simulink model "snap_sys_clk_feng"  (R2019a)
settings: Solver=VariableStepDiscrete  StartTime=0.0  StopTime=10.0  RelTol=1e-3
undefined symbols (not defined in the file): datetime, posixtime
libraries: xbsIndex_r4 x5252, casper_library_misc x69, xps_library x6, casper_library_delays x3
(part 15 of 45)

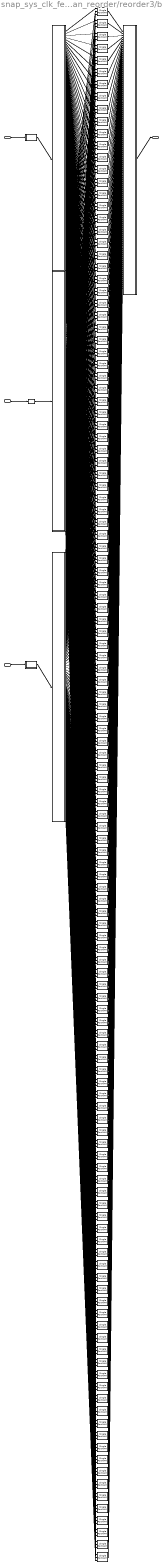
== system snap_sys_clk_feng/chan_reorder/reorder3/buf0 ==
  addr : Inport
  din : Inport  Port=2
  we : Inport  Port=3
  bram{0..127} (128 alike) : xbsIndex_r4/Single Port RAM  depth=16384  initVector=getfield(get_param(gcb, 'UserData'), 'initVector')  distributed_mem=Block RAM  write_mode=Read Before Write  rst=off  init_reg=0  en=off  latency=2  optimize=Speed  dbl_ovrd=off  block_type=spram
  ddin : xbsIndex_r4/Delay  rst=off  infoeditControl=Selection of Reset will increase slice count due to use of real FFs and instead of SRLs  en=off  latency=2  reg_retiming=on  dbl_ovrd=off  block_type=delay
  debus_addr : Subsystem  AncestorBlock=casper_library_flow_control/bus_expand  mask(bus_expand){mode=divisions of equal size, outputNum=128, outputWidth=[14 14 14 14 14 14 14 14 14 14 14 14 14 14 14 14 14 14 14 14 14 14 14 14 14 14 14 14 14 14 14 14 14 14 14 14 14 14 14 14 14 14 14 14 14 14 14 14 14 14 14 14 14 14 14 14 14 14 14 14 14 14 14 14 14 14 14 14 14 14 14 14 14 14 14 14 14 14 14 14 14 14 14 14 14 14 14 14 14 14 14 14 14 14 14 14 14 14 14 14 14 14 14 14 14 14 14 14 14 14 14 14 14 14 14 14 14 14 14 14 14 14 14 14 14 14 14 14], outputBinaryPt=[0 0 0 0 0 0 0 0 0 0 0 0 0 0 0 0 0 0 0 0 0 0 0 0 0 0 0 0 0 0 0 0 0 0 0 0 0 0 0 0 0 0 0 0 0 0 0 0 0 0 0 0 0 0 0 0 0 0 0 0 0 0 0 0 0 0 0 0 0 0 0 0 0 0 0 0 0 0 0 0 0 0 0 0 0 0 0 0 0 0 0 0 0 0 0 0 0 0 0 0 0 0 0 0 0 0 0 0 0 0 0 0 0 0 0 0 0 0 0 0 0 0 0 0 0 0 0 0], outputArithmeticType=[0 0 0 0 0 0 0 0 0 0 0 0 0 0 0 0 0 0 0 0 0 0 0 0 0 0 0 0 0 0 0 0 0 0 0 0 0 0 0 0 0 0 0 0 0 0 0 0 0 0 0 0 0 0 0 0 0 0 0 0 0 0 0 0 0 0 0 0 0 0 0 0 0 0 0 0 0 0 0 0 0 0 0 0 0 0 0 0 0 0 0 0 0 0 0 0 0 0 0 0 0 0 0 0 0 0 0 0 0 0 0 0 0 0 0 0 0 0 0 0 0 0 0 0 0 0 0 0], show_format=on, outputToWorkspace=off, variablePrefix=, outputToModelAsWell=on}
      mask prompts: outputNum "Number of outputs:"; outputWidth "Output width:"; outputBinaryPt "Output binary point position:"; outputArithmeticType "Output arithmetic type (ufix=0, fix=1, bool=2):"; show_format "Print format string?"; outputToWorkspace "Output to workspace?"; variablePrefix "Variable name prefix:"; outputToModelAsWell "Output to model as well?"
      mask help:
      | Expands a 'bus' made using a bus_create or Xilinx
      | concat block.
      | The input will be divided into the specified number
      | of outputs with the specified arithmetic types.
      | Divisions are made from most significant bit.
      mask init: same as snap_sys_clk_feng/corr/bus_expand
      settings: AttributesFormatString=128 outputs: uf14.0,uf14.0,uf14.0,uf14.0,uf14.0,uf14.0,uf14.0,uf14.0,uf14.0,uf14.0,uf14.0,uf14.0,uf14.0,uf14.0,uf14.0,uf14.0,uf14.0,uf14.0,uf14.0,uf14.0,uf14.0,uf14.0,uf14.0,uf14.0,uf14.0,uf14.0,uf14.0,uf14.0,uf14.0,uf14.0,uf14.0,uf14.0,uf14.0,uf14.0,uf14.0,uf14.0,uf14.0,uf14.0,uf14.0,uf14.0,uf14.0,uf14.0,uf14.0,uf14.0,uf14.0,uf14.0,uf14.0,uf14.0,uf14.0,uf14.0,uf14.0,uf14.0,uf14.0,uf14.0,uf14.0,uf14.0,uf14.0,uf14.0,uf14.0,uf14.0,uf14.0,uf14.0,uf14.0,uf14.0,uf14.0,uf14.0,uf14.0,uf14.0,uf14.0,uf14.0,uf14.0,uf14.0,uf14.0,uf14.0,uf14.0,uf14.0,uf14.0,uf14.0,uf14.0,uf14.0,uf14.0,uf14.0,uf14.0,uf14.0,uf14.0,uf14.0,uf14.0,uf14.0,uf14.0,uf14.0,uf14.0,uf14.0,uf14.0,uf14.0,uf14.0,uf14.0,uf14.0,uf14.0,uf14.0,uf14.0,uf14.0,uf14.0,uf14.0,uf14.0,uf14.0,uf14.0,uf14.0,uf14.0,uf14.0,uf14.0,uf14.0,uf14.0,uf14.0,uf14.0,uf14.0,uf14.0,uf14.0,uf14.0,uf14.0,uf14.0,uf14.0,uf14.0,uf14.0,uf14.0,uf14.0,uf14.0,uf14.0,uf14.0,
      mask TypeOptions mode: divisions of equal size | divisions of arbitrary size
      mask Callback mode: bus_expand_callback();
      mask Callback outputWidth: bus_expand_callback();
      mask Callback outputToWorkspace: bus_expand_callback();
  debus_din : Subsystem  AncestorBlock=casper_library_flow_control/bus_expand  mask(bus_expand){mode=divisions of arbitrary size, outputNum=1, outputWidth=[1 1 1 1 1 1 1 1 1 1 1 1 1 1 1 1 1 1 1 1 1 1 1 1 1 1 1 1 1 1 1 1 1 1 1 1 1 1 1 1 1 1 1 1 1 1 1 1 1 1 1 1 1 1 1 1 1 1 1 1 1 1 1 1 1 1 1 1 1 1 1 1 1 1 1 1 1 1 1 1 1 1 1 1 1 1 1 1 1 1 1 1 1 1 1 1 1 1 1 1 1 1 1 1 1 1 1 1 1 1 1 1 1 1 1 1 1 1 1 1 1 1 1 1 1 1 1 1], outputBinaryPt=[0 0 0 0 0 0 0 0 0 0 0 0 0 0 0 0 0 0 0 0 0 0 0 0 0 0 0 0 0 0 0 0 0 0 0 0 0 0 0 0 0 0 0 0 0 0 0 0 0 0 0 0 0 0 0 0 0 0 0 0 0 0 0 0 0 0 0 0 0 0 0 0 0 0 0 0 0 0 0 0 0 0 0 0 0 0 0 0 0 0 0 0 0 0 0 0 0 0 0 0 0 0 0 0 0 0 0 0 0 0 0 0 0 0 0 0 0 0 0 0 0 0 0 0 0 0 0 0], outputArithmeticType=[0 0 0 0 0 0 0 0 0 0 0 0 0 0 0 0 0 0 0 0 0 0 0 0 0 0 0 0 0 0 0 0 0 0 0 0 0 0 0 0 0 0 0 0 0 0 0 0 0 0 0 0 0 0 0 0 0 0 0 0 0 0 0 0 0 0 0 0 0 0 0 0 0 0 0 0 0 0 0 0 0 0 0 0 0 0 0 0 0 0 0 0 0 0 0 0 0 0 0 0 0 0 0 0 0 0 0 0 0 0 0 0 0 0 0 0 0 0 0 0 0 0 0 0 0 0 0 0], show_format=on, outputToWorkspace=off, variablePrefix=, outputToModelAsWell=on}
      mask prompts: outputNum "Number of outputs:"; outputWidth "Output width [msb ... lsb]:"; outputBinaryPt "Output binary point position [msb ... lsb]:"; outputArithmeticType "Output arithmetic type (ufix=0, fix=1, bool=2) [msb ... lsb]:"; show_format "Print format string?"; outputToWorkspace "Output to workspace?"; variablePrefix "Variable name prefix:"; outputToModelAsWell "Output to model as well?"
      mask help:
      | Expands a 'bus' made using a bus_create or Xilinx
      | concat block.
      | The input will be divided into the specified number
      | of outputs with the specified arithmetic types.
      | Divisions are made from most significant bit.
      mask init: same as snap_sys_clk_feng/corr/bus_expand
      settings: AttributesFormatString=128 outputs: uf1.0,uf1.0,uf1.0,uf1.0,uf1.0,uf1.0,uf1.0,uf1.0,uf1.0,uf1.0,uf1.0,uf1.0,uf1.0,uf1.0,uf1.0,uf1.0,uf1.0,uf1.0,uf1.0,uf1.0,uf1.0,uf1.0,uf1.0,uf1.0,uf1.0,uf1.0,uf1.0,uf1.0,uf1.0,uf1.0,uf1.0,uf1.0,uf1.0,uf1.0,uf1.0,uf1.0,uf1.0,uf1.0,uf1.0,uf1.0,uf1.0,uf1.0,uf1.0,uf1.0,uf1.0,uf1.0,uf1.0,uf1.0,uf1.0,uf1.0,uf1.0,uf1.0,uf1.0,uf1.0,uf1.0,uf1.0,uf1.0,uf1.0,uf1.0,uf1.0,uf1.0,uf1.0,uf1.0,uf1.0,uf1.0,uf1.0,uf1.0,uf1.0,uf1.0,uf1.0,uf1.0,uf1.0,uf1.0,uf1.0,uf1.0,uf1.0,uf1.0,uf1.0,uf1.0,uf1.0,uf1.0,uf1.0,uf1.0,uf1.0,uf1.0,uf1.0,uf1.0,uf1.0,uf1.0,uf1.0,uf1.0,uf1.0,uf1.0,uf1.0,uf1.0,uf1.0,uf1.0,uf1.0,uf1.0,uf1.0,uf1.0,uf1.0,uf1.0,uf1.0,uf1.0,uf1.0,uf1.0,uf1.0,uf1.0,uf1.0,uf1.0,uf1.0,uf1.0,uf1.0,uf1.0,uf1.0,uf1.0,uf1.0,uf1.0,uf1.0,uf1.0,uf1.0,uf1.0,uf1.0,uf1.0,uf1.0,uf1.0,uf1.0,
      mask TypeOptions mode: divisions of equal size | divisions of arbitrary size
      mask Callback mode: bus_expand_callback();
      mask Callback outputWidth: bus_expand_callback();
      mask Callback outputToWorkspace: bus_expand_callback();
  debus_we : Subsystem  AncestorBlock=casper_library_flow_control/bus_expand  mask(bus_expand){mode=divisions of equal size, outputNum=128, outputWidth=[1 1 1 1 1 1 1 1 1 1 1 1 1 1 1 1 1 1 1 1 1 1 1 1 1 1 1 1 1 1 1 1 1 1 1 1 1 1 1 1 1 1 1 1 1 1 1 1 1 1 1 1 1 1 1 1 1 1 1 1 1 1 1 1 1 1 1 1 1 1 1 1 1 1 1 1 1 1 1 1 1 1 1 1 1 1 1 1 1 1 1 1 1 1 1 1 1 1 1 1 1 1 1 1 1 1 1 1 1 1 1 1 1 1 1 1 1 1 1 1 1 1 1 1 1 1 1 1], outputBinaryPt=[0 0 0 0 0 0 0 0 0 0 0 0 0 0 0 0 0 0 0 0 0 0 0 0 0 0 0 0 0 0 0 0 0 0 0 0 0 0 0 0 0 0 0 0 0 0 0 0 0 0 0 0 0 0 0 0 0 0 0 0 0 0 0 0 0 0 0 0 0 0 0 0 0 0 0 0 0 0 0 0 0 0 0 0 0 0 0 0 0 0 0 0 0 0 0 0 0 0 0 0 0 0 0 0 0 0 0 0 0 0 0 0 0 0 0 0 0 0 0 0 0 0 0 0 0 0 0 0], outputArithmeticType=[2 2 2 2 2 2 2 2 2 2 2 2 2 2 2 2 2 2 2 2 2 2 2 2 2 2 2 2 2 2 2 2 2 2 2 2 2 2 2 2 2 2 2 2 2 2 2 2 2 2 2 2 2 2 2 2 2 2 2 2 2 2 2 2 2 2 2 2 2 2 2 2 2 2 2 2 2 2 2 2 2 2 2 2 2 2 2 2 2 2 2 2 2 2 2 2 2 2 2 2 2 2 2 2 2 2 2 2 2 2 2 2 2 2 2 2 2 2 2 2 2 2 2 2 2 2 2 2], show_format=on, outputToWorkspace=off, variablePrefix=, outputToModelAsWell=on}
      mask prompts: outputNum "Number of outputs:"; outputWidth "Output width:"; outputBinaryPt "Output binary point position:"; outputArithmeticType "Output arithmetic type (ufix=0, fix=1, bool=2):"; show_format "Print format string?"; outputToWorkspace "Output to workspace?"; variablePrefix "Variable name prefix:"; outputToModelAsWell "Output to model as well?"
      mask help:
      | Expands a 'bus' made using a bus_create or Xilinx
      | concat block.
      | The input will be divided into the specified number
      | of outputs with the specified arithmetic types.
      | Divisions are made from most significant bit.
      mask init: same as snap_sys_clk_feng/corr/bus_expand
      settings: AttributesFormatString=128 outputs: b,b,b,b,b,b,b,b,b,b,b,b,b,b,b,b,b,b,b,b,b,b,b,b,b,b,b,b,b,b,b,b,b,b,b,b,b,b,b,b,b,b,b,b,b,b,b,b,b,b,b,b,b,b,b,b,b,b,b,b,b,b,b,b,b,b,b,b,b,b,b,b,b,b,b,b,b,b,b,b,b,b,b,b,b,b,b,b,b,b,b,b,b,b,b,b,b,b,b,b,b,b,b,b,b,b,b,b,b,b,b,b,b,b,b,b,b,b,b,b,b,b,b,b,b,b,b,b,
      mask TypeOptions mode: divisions of equal size | divisions of arbitrary size
      mask Callback mode: bus_expand_callback();
      mask Callback outputWidth: bus_expand_callback();
      mask Callback outputToWorkspace: bus_expand_callback();
  din_bussify : Subsystem  AncestorBlock=casper_library_flow_control/bus_create  mask(bus_create){inputNum=128}
      mask prompts: inputNum "Number of inputs:"
      mask init:
      | bus_create_init(gcb,...
      |     'inputNum', inputNum);
  rep_addr : Subsystem  AncestorBlock=casper_library_bus/bus_replicate  mask(bus_replicate){replication=128, csp_latency=2, misc=off, implementation=core}
      mask prompts: replication "replication factor"; csp_latency "latency"; misc "misc support"; implementation "delay implementation"
      mask help: Output bus formed by replicating input bus a number of times
      mask init:
      | bus_replicate_init(gcb, ...
      |     'replication', replication, ...
      |     'csp_latency', csp_latency, ...
      |     'implementation', implementation, ...
      |     'misc', misc);
      mask TypeOptions implementation: core | behavioral
  rep_we : Subsystem  AncestorBlock=casper_library_bus/bus_replicate  mask(bus_replicate){replication=128, csp_latency=2, misc=off, implementation=core}
      mask prompts: replication "replication factor"; csp_latency "latency"; misc "misc support"; implementation "delay implementation"
      mask help: Output bus formed by replicating input bus a number of times
      mask init:
      | bus_replicate_init(gcb, ...
      |     'replication', replication, ...
      |     'csp_latency', csp_latency, ...
      |     'implementation', implementation, ...
      |     'misc', misc);
      mask TypeOptions implementation: core | behavioral
  dout : Outport
  wires:
  addr/1 -> rep_addr/1(in)
  din/1 -> ddin/1
  we/1 -> rep_we/1(in)
  rep_addr/1(out) -> debus_addr/1(bus_in)
  ddin/1 -> debus_din/1(bus_in)
  rep_we/1(out) -> debus_we/1(bus_in)
  debus_addr/1(msb_out128) -> bram0/1
  debus_din/1(msb_out128) -> bram0/2
  debus_we/1(msb_out128) -> bram0/3
  debus_addr/2(out127) -> bram1/1
  debus_din/2(out127) -> bram1/2
  debus_we/2(out127) -> bram1/3
  debus_addr/3(out126) -> bram2/1
  debus_din/3(out126) -> bram2/2
  debus_we/3(out126) -> bram2/3
  debus_addr/4(out125) -> bram3/1
  debus_din/4(out125) -> bram3/2
  debus_we/4(out125) -> bram3/3
  debus_addr/5(out124) -> bram4/1
  debus_din/5(out124) -> bram4/2
  debus_we/5(out124) -> bram4/3
  debus_addr/6(out123) -> bram5/1
  debus_din/6(out123) -> bram5/2
  debus_we/6(out123) -> bram5/3
  debus_addr/7(out122) -> bram6/1
  debus_din/7(out122) -> bram6/2
  debus_we/7(out122) -> bram6/3
  debus_addr/8(out121) -> bram7/1
  debus_din/8(out121) -> bram7/2
  debus_we/8(out121) -> bram7/3
  debus_addr/9(out120) -> bram8/1
  debus_din/9(out120) -> bram8/2
  debus_we/9(out120) -> bram8/3
  debus_addr/10(out119) -> bram9/1
  debus_din/10(out119) -> bram9/2
  debus_we/10(out119) -> bram9/3
  debus_addr/11(out118) -> bram10/1
  debus_din/11(out118) -> bram10/2
  debus_we/11(out118) -> bram10/3
  debus_addr/12(out117) -> bram11/1
  debus_din/12(out117) -> bram11/2
  debus_we/12(out117) -> bram11/3
  debus_addr/13(out116) -> bram12/1
  debus_din/13(out116) -> bram12/2
  debus_we/13(out116) -> bram12/3
  debus_addr/14(out115) -> bram13/1
  debus_din/14(out115) -> bram13/2
  debus_we/14(out115) -> bram13/3
  debus_addr/15(out114) -> bram14/1
  debus_din/15(out114) -> bram14/2
  debus_we/15(out114) -> bram14/3
  debus_addr/16(out113) -> bram15/1
  debus_din/16(out113) -> bram15/2
  debus_we/16(out113) -> bram15/3
  debus_addr/17(out112) -> bram16/1
  debus_din/17(out112) -> bram16/2
  debus_we/17(out112) -> bram16/3
  debus_addr/18(out111) -> bram17/1
  debus_din/18(out111) -> bram17/2
  debus_we/18(out111) -> bram17/3
  debus_addr/19(out110) -> bram18/1
  debus_din/19(out110) -> bram18/2
  debus_we/19(out110) -> bram18/3
  debus_addr/20(out109) -> bram19/1
  debus_din/20(out109) -> bram19/2
  debus_we/20(out109) -> bram19/3
  debus_addr/21(out108) -> bram20/1
  debus_din/21(out108) -> bram20/2
  debus_we/21(out108) -> bram20/3
  debus_addr/22(out107) -> bram21/1
  debus_din/22(out107) -> bram21/2
  debus_we/22(out107) -> bram21/3
  debus_addr/23(out106) -> bram22/1
  debus_din/23(out106) -> bram22/2
  debus_we/23(out106) -> bram22/3
  debus_addr/24(out105) -> bram23/1
  debus_din/24(out105) -> bram23/2
  debus_we/24(out105) -> bram23/3
  debus_addr/25(out104) -> bram24/1
  debus_din/25(out104) -> bram24/2
  debus_we/25(out104) -> bram24/3
  debus_addr/26(out103) -> bram25/1
  debus_din/26(out103) -> bram25/2
  debus_we/26(out103) -> bram25/3
  debus_addr/27(out102) -> bram26/1
  debus_din/27(out102) -> bram26/2
  debus_we/27(out102) -> bram26/3
  debus_addr/28(out101) -> bram27/1
  debus_din/28(out101) -> bram27/2
  debus_we/28(out101) -> bram27/3
  debus_addr/29(out100) -> bram28/1
  debus_din/29(out100) -> bram28/2
  debus_we/29(out100) -> bram28/3
  debus_addr/30(out99) -> bram29/1
  debus_din/30(out99) -> bram29/2
  debus_we/30(out99) -> bram29/3
  debus_addr/31(out98) -> bram30/1
  debus_din/31(out98) -> bram30/2
  debus_we/31(out98) -> bram30/3
  debus_addr/32(out97) -> bram31/1
  debus_din/32(out97) -> bram31/2
  debus_we/32(out97) -> bram31/3
  debus_addr/33(out96) -> bram32/1
  debus_din/33(out96) -> bram32/2
  debus_we/33(out96) -> bram32/3
  debus_addr/34(out95) -> bram33/1
  debus_din/34(out95) -> bram33/2
  debus_we/34(out95) -> bram33/3
  debus_addr/35(out94) -> bram34/1
  debus_din/35(out94) -> bram34/2
  debus_we/35(out94) -> bram34/3
  debus_addr/36(out93) -> bram35/1
  debus_din/36(out93) -> bram35/2
  debus_we/36(out93) -> bram35/3
  debus_addr/37(out92) -> bram36/1
  debus_din/37(out92) -> bram36/2
  debus_we/37(out92) -> bram36/3
  debus_addr/38(out91) -> bram37/1
  debus_din/38(out91) -> bram37/2
  debus_we/38(out91) -> bram37/3
  debus_addr/39(out90) -> bram38/1
  debus_din/39(out90) -> bram38/2
  debus_we/39(out90) -> bram38/3
  debus_addr/40(out89) -> bram39/1
  debus_din/40(out89) -> bram39/2
  debus_we/40(out89) -> bram39/3
  debus_addr/41(out88) -> bram40/1
  debus_din/41(out88) -> bram40/2
  debus_we/41(out88) -> bram40/3
  debus_addr/42(out87) -> bram41/1
  debus_din/42(out87) -> bram41/2
  debus_we/42(out87) -> bram41/3
  debus_addr/43(out86) -> bram42/1
  debus_din/43(out86) -> bram42/2
  debus_we/43(out86) -> bram42/3
  debus_addr/44(out85) -> bram43/1
  debus_din/44(out85) -> bram43/2
  debus_we/44(out85) -> bram43/3
  debus_addr/45(out84) -> bram44/1
  debus_din/45(out84) -> bram44/2
  debus_we/45(out84) -> bram44/3
  debus_addr/46(out83) -> bram45/1
  debus_din/46(out83) -> bram45/2
  debus_we/46(out83) -> bram45/3
  debus_addr/47(out82) -> bram46/1
  debus_din/47(out82) -> bram46/2
  debus_we/47(out82) -> bram46/3
  debus_addr/48(out81) -> bram47/1
  debus_din/48(out81) -> bram47/2
  debus_we/48(out81) -> bram47/3
  debus_addr/49(out80) -> bram48/1
  debus_din/49(out80) -> bram48/2
  debus_we/49(out80) -> bram48/3
  debus_addr/50(out79) -> bram49/1
  debus_din/50(out79) -> bram49/2
  debus_we/50(out79) -> bram49/3
  debus_addr/51(out78) -> bram50/1
  debus_din/51(out78) -> bram50/2
  debus_we/51(out78) -> bram50/3
  debus_addr/52(out77) -> bram51/1
  debus_din/52(out77) -> bram51/2
  debus_we/52(out77) -> bram51/3
  debus_addr/53(out76) -> bram52/1
  debus_din/53(out76) -> bram52/2
  debus_we/53(out76) -> bram52/3
  debus_addr/54(out75) -> bram53/1
  debus_din/54(out75) -> bram53/2
  debus_we/54(out75) -> bram53/3
  debus_addr/55(out74) -> bram54/1
  debus_din/55(out74) -> bram54/2
  debus_we/55(out74) -> bram54/3
  debus_addr/56(out73) -> bram55/1
  debus_din/56(out73) -> bram55/2
  debus_we/56(out73) -> bram55/3
  debus_addr/57(out72) -> bram56/1
  debus_din/57(out72) -> bram56/2
  debus_we/57(out72) -> bram56/3
  debus_addr/58(out71) -> bram57/1
  debus_din/58(out71) -> bram57/2
  debus_we/58(out71) -> bram57/3
  debus_addr/59(out70) -> bram58/1
  debus_din/59(out70) -> bram58/2
  debus_we/59(out70) -> bram58/3
  debus_addr/60(out69) -> bram59/1
  debus_din/60(out69) -> bram59/2
  debus_we/60(out69) -> bram59/3
  debus_addr/61(out68) -> bram60/1
  debus_din/61(out68) -> bram60/2
  debus_we/61(out68) -> bram60/3
  debus_addr/62(out67) -> bram61/1
  debus_din/62(out67) -> bram61/2
  debus_we/62(out67) -> bram61/3
  debus_addr/63(out66) -> bram62/1
  debus_din/63(out66) -> bram62/2
  debus_we/63(out66) -> bram62/3
  debus_addr/64(out65) -> bram63/1
  debus_din/64(out65) -> bram63/2
  debus_we/64(out65) -> bram63/3
  debus_addr/65(out64) -> bram64/1
  debus_din/65(out64) -> bram64/2
  debus_we/65(out64) -> bram64/3
  debus_addr/66(out63) -> bram65/1
  debus_din/66(out63) -> bram65/2
  debus_we/66(out63) -> bram65/3
  debus_addr/67(out62) -> bram66/1
  debus_din/67(out62) -> bram66/2
  debus_we/67(out62) -> bram66/3
  debus_addr/68(out61) -> bram67/1
  debus_din/68(out61) -> bram67/2
  debus_we/68(out61) -> bram67/3
  debus_addr/69(out60) -> bram68/1
  debus_din/69(out60) -> bram68/2
  debus_we/69(out60) -> bram68/3
  debus_addr/70(out59) -> bram69/1
  debus_din/70(out59) -> bram69/2
  debus_we/70(out59) -> bram69/3
  debus_addr/71(out58) -> bram70/1
  debus_din/71(out58) -> bram70/2
  debus_we/71(out58) -> bram70/3
  debus_addr/72(out57) -> bram71/1
  debus_din/72(out57) -> bram71/2
  debus_we/72(out57) -> bram71/3
  debus_addr/73(out56) -> bram72/1
  debus_din/73(out56) -> bram72/2
  debus_we/73(out56) -> bram72/3
  debus_addr/74(out55) -> bram73/1
  debus_din/74(out55) -> bram73/2
  debus_we/74(out55) -> bram73/3
  debus_addr/75(out54) -> bram74/1
  debus_din/75(out54) -> bram74/2
  debus_we/75(out54) -> bram74/3
  debus_addr/76(out53) -> bram75/1
  debus_din/76(out53) -> bram75/2
  debus_we/76(out53) -> bram75/3
  debus_addr/77(out52) -> bram76/1
  debus_din/77(out52) -> bram76/2
  debus_we/77(out52) -> bram76/3
  debus_addr/78(out51) -> bram77/1
  debus_din/78(out51) -> bram77/2
  debus_we/78(out51) -> bram77/3
  debus_addr/79(out50) -> bram78/1
  debus_din/79(out50) -> bram78/2
  debus_we/79(out50) -> bram78/3
  debus_addr/80(out49) -> bram79/1
  debus_din/80(out49) -> bram79/2
  debus_we/80(out49) -> bram79/3
  debus_addr/81(out48) -> bram80/1
  debus_din/81(out48) -> bram80/2
  debus_we/81(out48) -> bram80/3
  debus_addr/82(out47) -> bram81/1
  debus_din/82(out47) -> bram81/2
  debus_we/82(out47) -> bram81/3
  debus_addr/83(out46) -> bram82/1
  debus_din/83(out46) -> bram82/2
  debus_we/83(out46) -> bram82/3
  debus_addr/84(out45) -> bram83/1
  debus_din/84(out45) -> bram83/2
  debus_we/84(out45) -> bram83/3
  debus_addr/85(out44) -> bram84/1
  debus_din/85(out44) -> bram84/2
  debus_we/85(out44) -> bram84/3
  debus_addr/86(out43) -> bram85/1
  debus_din/86(out43) -> bram85/2
  debus_we/86(out43) -> bram85/3
  debus_addr/87(out42) -> bram86/1
  debus_din/87(out42) -> bram86/2
  debus_we/87(out42) -> bram86/3
  debus_addr/88(out41) -> bram87/1
  debus_din/88(out41) -> bram87/2
  debus_we/88(out41) -> bram87/3
  debus_addr/89(out40) -> bram88/1
  debus_din/89(out40) -> bram88/2
  debus_we/89(out40) -> bram88/3
  debus_addr/90(out39) -> bram89/1
  debus_din/90(out39) -> bram89/2
  debus_we/90(out39) -> bram89/3
  debus_addr/91(out38) -> bram90/1
  debus_din/91(out38) -> bram90/2
  debus_we/91(out38) -> bram90/3
  debus_addr/92(out37) -> bram91/1
  debus_din/92(out37) -> bram91/2
  debus_we/92(out37) -> bram91/3
  debus_addr/93(out36) -> bram92/1
  debus_din/93(out36) -> bram92/2
  debus_we/93(out36) -> bram92/3
  debus_addr/94(out35) -> bram93/1
  debus_din/94(out35) -> bram93/2
  debus_we/94(out35) -> bram93/3
  debus_addr/95(out34) -> bram94/1
  debus_din/95(out34) -> bram94/2
  debus_we/95(out34) -> bram94/3
  debus_addr/96(out33) -> bram95/1
  debus_din/96(out33) -> bram95/2
  debus_we/96(out33) -> bram95/3
  debus_addr/97(out32) -> bram96/1
  debus_din/97(out32) -> bram96/2
  debus_we/97(out32) -> bram96/3
  debus_addr/98(out31) -> bram97/1
  debus_din/98(out31) -> bram97/2
  debus_we/98(out31) -> bram97/3
  debus_addr/99(out30) -> bram98/1
  debus_din/99(out30) -> bram98/2
  debus_we/99(out30) -> bram98/3
  debus_addr/100(out29) -> bram99/1
  debus_din/100(out29) -> bram99/2
  debus_we/100(out29) -> bram99/3
  debus_addr/101(out28) -> bram100/1
  debus_din/101(out28) -> bram100/2
  debus_we/101(out28) -> bram100/3
  debus_addr/102(out27) -> bram101/1
  debus_din/102(out27) -> bram101/2
  debus_we/102(out27) -> bram101/3
  debus_addr/103(out26) -> bram102/1
  debus_din/103(out26) -> bram102/2
  debus_we/103(out26) -> bram102/3
  debus_addr/104(out25) -> bram103/1
  debus_din/104(out25) -> bram103/2
  debus_we/104(out25) -> bram103/3
  debus_addr/105(out24) -> bram104/1
  debus_din/105(out24) -> bram104/2
  debus_we/105(out24) -> bram104/3
  debus_addr/106(out23) -> bram105/1
  debus_din/106(out23) -> bram105/2
  debus_we/106(out23) -> bram105/3
  debus_addr/107(out22) -> bram106/1
  debus_din/107(out22) -> bram106/2
  debus_we/107(out22) -> bram106/3
  debus_addr/108(out21) -> bram107/1
  debus_din/108(out21) -> bram107/2
  debus_we/108(out21) -> bram107/3
  debus_addr/109(out20) -> bram108/1
  debus_din/109(out20) -> bram108/2
  debus_we/109(out20) -> bram108/3
  debus_addr/110(out19) -> bram109/1
  debus_din/110(out19) -> bram109/2
  debus_we/110(out19) -> bram109/3
  debus_addr/111(out18) -> bram110/1
  debus_din/111(out18) -> bram110/2
  debus_we/111(out18) -> bram110/3
  debus_addr/112(out17) -> bram111/1
  debus_din/112(out17) -> bram111/2
  debus_we/112(out17) -> bram111/3
  debus_addr/113(out16) -> bram112/1
  debus_din/113(out16) -> bram112/2
  debus_we/113(out16) -> bram112/3
  debus_addr/114(out15) -> bram113/1
  debus_din/114(out15) -> bram113/2
  debus_we/114(out15) -> bram113/3
  debus_addr/115(out14) -> bram114/1
  debus_din/115(out14) -> bram114/2
  debus_we/115(out14) -> bram114/3
  debus_addr/116(out13) -> bram115/1
  debus_din/116(out13) -> bram115/2
  debus_we/116(out13) -> bram115/3
  debus_addr/117(out12) -> bram116/1
  debus_din/117(out12) -> bram116/2
  debus_we/117(out12) -> bram116/3
  debus_addr/118(out11) -> bram117/1
  debus_din/118(out11) -> bram117/2
  debus_we/118(out11) -> bram117/3
  debus_addr/119(out10) -> bram118/1
  debus_din/119(out10) -> bram118/2
  debus_we/119(out10) -> bram118/3
  debus_addr/120(out9) -> bram119/1
  debus_din/120(out9) -> bram119/2
  debus_we/120(out9) -> bram119/3
  debus_addr/121(out8) -> bram120/1
  debus_din/121(out8) -> bram120/2
  debus_we/121(out8) -> bram120/3
  debus_addr/122(out7) -> bram121/1
  debus_din/122(out7) -> bram121/2
  debus_we/122(out7) -> bram121/3
  debus_addr/123(out6) -> bram122/1
  debus_din/123(out6) -> bram122/2
  debus_we/123(out6) -> bram122/3
  debus_addr/124(out5) -> bram123/1
  debus_din/124(out5) -> bram123/2
  debus_we/124(out5) -> bram123/3
  debus_addr/125(out4) -> bram124/1
  debus_din/125(out4) -> bram124/2
  debus_we/125(out4) -> bram124/3
  debus_addr/126(out3) -> bram125/1
  debus_din/126(out3) -> bram125/2
  debus_we/126(out3) -> bram125/3
  debus_addr/127(out2) -> bram126/1
  debus_din/127(out2) -> bram126/2
  debus_we/127(out2) -> bram126/3
  debus_addr/128(lsb_out1) -> bram127/1
  debus_din/128(lsb_out1) -> bram127/2
  debus_we/128(lsb_out1) -> bram127/3
  bram0/1 -> din_bussify/1(in1)
  bram1/1 -> din_bussify/2(in2)
  bram2/1 -> din_bussify/3(in3)
  bram3/1 -> din_bussify/4(in4)
  bram4/1 -> din_bussify/5(in5)
  bram5/1 -> din_bussify/6(in6)
  bram6/1 -> din_bussify/7(in7)
  bram7/1 -> din_bussify/8(in8)
  bram8/1 -> din_bussify/9(in9)
  bram9/1 -> din_bussify/10(in10)
  bram10/1 -> din_bussify/11(in11)
  bram11/1 -> din_bussify/12(in12)
  bram12/1 -> din_bussify/13(in13)
  bram13/1 -> din_bussify/14(in14)
  bram14/1 -> din_bussify/15(in15)
  bram15/1 -> din_bussify/16(in16)
  bram16/1 -> din_bussify/17(in17)
  bram17/1 -> din_bussify/18(in18)
  bram18/1 -> din_bussify/19(in19)
  bram19/1 -> din_bussify/20(in20)
  bram20/1 -> din_bussify/21(in21)
  bram21/1 -> din_bussify/22(in22)
  bram22/1 -> din_bussify/23(in23)
  bram23/1 -> din_bussify/24(in24)
  bram24/1 -> din_bussify/25(in25)
  bram25/1 -> din_bussify/26(in26)
  bram26/1 -> din_bussify/27(in27)
  bram27/1 -> din_bussify/28(in28)
  bram28/1 -> din_bussify/29(in29)
  bram29/1 -> din_bussify/30(in30)
  bram30/1 -> din_bussify/31(in31)
  bram31/1 -> din_bussify/32(in32)
  bram32/1 -> din_bussify/33(in33)
  bram33/1 -> din_bussify/34(in34)
  bram34/1 -> din_bussify/35(in35)
  bram35/1 -> din_bussify/36(in36)
  bram36/1 -> din_bussify/37(in37)
  bram37/1 -> din_bussify/38(in38)
  bram38/1 -> din_bussify/39(in39)
  bram39/1 -> din_bussify/40(in40)
  bram40/1 -> din_bussify/41(in41)
  bram41/1 -> din_bussify/42(in42)
  bram42/1 -> din_bussify/43(in43)
  bram43/1 -> din_bussify/44(in44)
  bram44/1 -> din_bussify/45(in45)
  bram45/1 -> din_bussify/46(in46)
  bram46/1 -> din_bussify/47(in47)
  bram47/1 -> din_bussify/48(in48)
  bram48/1 -> din_bussify/49(in49)
  bram49/1 -> din_bussify/50(in50)
  bram50/1 -> din_bussify/51(in51)
  bram51/1 -> din_bussify/52(in52)
  bram52/1 -> din_bussify/53(in53)
  bram53/1 -> din_bussify/54(in54)
  bram54/1 -> din_bussify/55(in55)
  bram55/1 -> din_bussify/56(in56)
  bram56/1 -> din_bussify/57(in57)
  bram57/1 -> din_bussify/58(in58)
  bram58/1 -> din_bussify/59(in59)
  bram59/1 -> din_bussify/60(in60)
  bram60/1 -> din_bussify/61(in61)
  bram61/1 -> din_bussify/62(in62)
  bram62/1 -> din_bussify/63(in63)
  bram63/1 -> din_bussify/64(in64)
  bram64/1 -> din_bussify/65(in65)
  bram65/1 -> din_bussify/66(in66)
  bram66/1 -> din_bussify/67(in67)
  bram67/1 -> din_bussify/68(in68)
  bram68/1 -> din_bussify/69(in69)
  bram69/1 -> din_bussify/70(in70)
  bram70/1 -> din_bussify/71(in71)
  bram71/1 -> din_bussify/72(in72)
  bram72/1 -> din_bussify/73(in73)
  bram73/1 -> din_bussify/74(in74)
  bram74/1 -> din_bussify/75(in75)
  bram75/1 -> din_bussify/76(in76)
  bram76/1 -> din_bussify/77(in77)
  bram77/1 -> din_bussify/78(in78)
  bram78/1 -> din_bussify/79(in79)
  bram79/1 -> din_bussify/80(in80)
  bram80/1 -> din_bussify/81(in81)
  bram81/1 -> din_bussify/82(in82)
  bram82/1 -> din_bussify/83(in83)
  bram83/1 -> din_bussify/84(in84)
  bram84/1 -> din_bussify/85(in85)
  bram85/1 -> din_bussify/86(in86)
  bram86/1 -> din_bussify/87(in87)
  bram87/1 -> din_bussify/88(in88)
  bram88/1 -> din_bussify/89(in89)
  bram89/1 -> din_bussify/90(in90)
  bram90/1 -> din_bussify/91(in91)
  bram91/1 -> din_bussify/92(in92)
  bram92/1 -> din_bussify/93(in93)
  bram93/1 -> din_bussify/94(in94)
  bram94/1 -> din_bussify/95(in95)
  bram95/1 -> din_bussify/96(in96)
  bram96/1 -> din_bussify/97(in97)
  bram97/1 -> din_bussify/98(in98)
  bram98/1 -> din_bussify/99(in99)
  bram99/1 -> din_bussify/100(in100)
  bram100/1 -> din_bussify/101(in101)
  bram101/1 -> din_bussify/102(in102)
  bram102/1 -> din_bussify/103(in103)
  bram103/1 -> din_bussify/104(in104)
  bram104/1 -> din_bussify/105(in105)
  bram105/1 -> din_bussify/106(in106)
  bram106/1 -> din_bussify/107(in107)
  bram107/1 -> din_bussify/108(in108)
  bram108/1 -> din_bussify/109(in109)
  bram109/1 -> din_bussify/110(in110)
  bram110/1 -> din_bussify/111(in111)
  bram111/1 -> din_bussify/112(in112)
  bram112/1 -> din_bussify/113(in113)
  bram113/1 -> din_bussify/114(in114)
  bram114/1 -> din_bussify/115(in115)
  bram115/1 -> din_bussify/116(in116)
  bram116/1 -> din_bussify/117(in117)
  bram117/1 -> din_bussify/118(in118)
  bram118/1 -> din_bussify/119(in119)
  bram119/1 -> din_bussify/120(in120)
  bram120/1 -> din_bussify/121(in121)
  bram121/1 -> din_bussify/122(in122)
  bram122/1 -> din_bussify/123(in123)
  bram123/1 -> din_bussify/124(in124)
  bram124/1 -> din_bussify/125(in125)
  bram125/1 -> din_bussify/126(in126)
  bram126/1 -> din_bussify/127(in127)
  bram127/1 -> din_bussify/128(in128)
  din_bussify/1(bus_out) -> dout/1

== system snap_sys_clk_feng/chan_reorder/reorder3/current_map ==
  addra : Inport
  dina : Inport  Port=2
  wea : Inport  Port=3
  addrb : Inport  Port=4
  dinb : Inport  Port=5
  web : Inport  Port=6
  A_bussify0 : Subsystem  AncestorBlock=casper_library_flow_control/bus_create  mask(bus_create){inputNum=7}
      mask prompts: inputNum "Number of inputs:"
      mask init:
      | bus_create_init(gcb,...
      |     'inputNum', inputNum);
  B_bussify0 : Subsystem  AncestorBlock=casper_library_flow_control/bus_create  mask(bus_create){inputNum=7}
      mask prompts: inputNum "Number of inputs:"
      mask init:
      | bus_create_init(gcb,...
      |     'inputNum', inputNum);
  alsbs_slice : xbsIndex_r4/Slice  nbits=14  boolean_output=off  mode=Lower Bit Location + Width  bit1=0  base1=LSB of Input  bit0=0  base0=LSB of Input  dbl_ovrd=off  block_type=slice
  blsbs_slice : xbsIndex_r4/Slice  nbits=14  boolean_output=off  mode=Lower Bit Location + Width  bit1=0  base1=LSB of Input  bit0=0  base0=LSB of Input  dbl_ovrd=off  block_type=slice
  bram0_{0..6} (7 alike) : xbsIndex_r4/Dual Port RAM  depth=16384  initVector=getfield(get_param(gcb, 'UserData'), 'initVector')  distributed_mem=Block RAM  init_a=0  init_b=0  rst_a=off  rst_b=off  en_a=off  en_b=off  latency=2  write_mode_A=Read Before Write  write_mode_B=Read Before Write  optimize=Speed  dbl_ovrd=off  block_type=dpram
  ddina0 : xbsIndex_r4/Delay  rst=off  infoeditControl=Selection of Reset will increase slice count due to use of real FFs and instead of SRLs  en=off  latency=0  reg_retiming=on  dbl_ovrd=off  block_type=delay
  ddinb0 : xbsIndex_r4/Delay  rst=off  infoeditControl=Selection of Reset will increase slice count due to use of real FFs and instead of SRLs  en=off  latency=0  reg_retiming=on  dbl_ovrd=off  block_type=delay
  debus_addra0 : Subsystem  AncestorBlock=casper_library_flow_control/bus_expand  mask(bus_expand){mode=divisions of equal size, outputNum=7, outputWidth=[14 14 14 14 14 14 14], outputBinaryPt=[0 0 0 0 0 0 0], outputArithmeticType=[0 0 0 0 0 0 0], show_format=on, outputToWorkspace=off, variablePrefix=, outputToModelAsWell=on}
      mask prompts: outputNum "Number of outputs:"; outputWidth "Output width:"; outputBinaryPt "Output binary point position:"; outputArithmeticType "Output arithmetic type (ufix=0, fix=1, bool=2):"; show_format "Print format string?"; outputToWorkspace "Output to workspace?"; variablePrefix "Variable name prefix:"; outputToModelAsWell "Output to model as well?"
      mask help:
      | Expands a 'bus' made using a bus_create or Xilinx
      | concat block.
      | The input will be divided into the specified number
      | of outputs with the specified arithmetic types.
      | Divisions are made from most significant bit.
      mask init: same as snap_sys_clk_feng/corr/bus_expand
      settings: AttributesFormatString=7 outputs: uf14.0,uf14.0,uf14.0,uf14.0,uf14.0,uf14.0,uf14.0,
      mask TypeOptions mode: divisions of equal size | divisions of arbitrary size
      mask Callback mode: bus_expand_callback();
      mask Callback outputWidth: bus_expand_callback();
      mask Callback outputToWorkspace: bus_expand_callback();
  debus_addrb0 : Subsystem  AncestorBlock=casper_library_flow_control/bus_expand  mask(bus_expand){mode=divisions of equal size, outputNum=7, outputWidth=[14 14 14 14 14 14 14], outputBinaryPt=[0 0 0 0 0 0 0], outputArithmeticType=[0 0 0 0 0 0 0], show_format=on, outputToWorkspace=off, variablePrefix=, outputToModelAsWell=on}
      mask prompts: outputNum "Number of outputs:"; outputWidth "Output width:"; outputBinaryPt "Output binary point position:"; outputArithmeticType "Output arithmetic type (ufix=0, fix=1, bool=2):"; show_format "Print format string?"; outputToWorkspace "Output to workspace?"; variablePrefix "Variable name prefix:"; outputToModelAsWell "Output to model as well?"
      mask help:
      | Expands a 'bus' made using a bus_create or Xilinx
      | concat block.
      | The input will be divided into the specified number
      | of outputs with the specified arithmetic types.
      | Divisions are made from most significant bit.
      mask init: same as snap_sys_clk_feng/corr/bus_expand
      settings: AttributesFormatString=7 outputs: uf14.0,uf14.0,uf14.0,uf14.0,uf14.0,uf14.0,uf14.0,
      mask TypeOptions mode: divisions of equal size | divisions of arbitrary size
      mask Callback mode: bus_expand_callback();
      mask Callback outputWidth: bus_expand_callback();
      mask Callback outputToWorkspace: bus_expand_callback();
  debus_dina0 : Subsystem  AncestorBlock=casper_library_flow_control/bus_expand  mask(bus_expand){mode=divisions of arbitrary size, outputNum=1, outputWidth=[2 2 2 2 2 2 2], outputBinaryPt=[0 0 0 0 0 0 0], outputArithmeticType=[0 0 0 0 0 0 0], show_format=on, outputToWorkspace=off, variablePrefix=, outputToModelAsWell=on}
      mask prompts: outputNum "Number of outputs:"; outputWidth "Output width [msb ... lsb]:"; outputBinaryPt "Output binary point position [msb ... lsb]:"; outputArithmeticType "Output arithmetic type (ufix=0, fix=1, bool=2) [msb ... lsb]:"; show_format "Print format string?"; outputToWorkspace "Output to workspace?"; variablePrefix "Variable name prefix:"; outputToModelAsWell "Output to model as well?"
      mask help:
      | Expands a 'bus' made using a bus_create or Xilinx
      | concat block.
      | The input will be divided into the specified number
      | of outputs with the specified arithmetic types.
      | Divisions are made from most significant bit.
      mask init: same as snap_sys_clk_feng/corr/bus_expand
      settings: AttributesFormatString=7 outputs: uf2.0,uf2.0,uf2.0,uf2.0,uf2.0,uf2.0,uf2.0,
      mask TypeOptions mode: divisions of equal size | divisions of arbitrary size
      mask Callback mode: bus_expand_callback();
      mask Callback outputWidth: bus_expand_callback();
      mask Callback outputToWorkspace: bus_expand_callback();
  debus_dinb0 : Subsystem  AncestorBlock=casper_library_flow_control/bus_expand  mask(bus_expand){mode=divisions of arbitrary size, outputNum=1, outputWidth=[2 2 2 2 2 2 2], outputBinaryPt=[0 0 0 0 0 0 0], outputArithmeticType=[0 0 0 0 0 0 0], show_format=on, outputToWorkspace=off, variablePrefix=, outputToModelAsWell=on}
      mask prompts: outputNum "Number of outputs:"; outputWidth "Output width [msb ... lsb]:"; outputBinaryPt "Output binary point position [msb ... lsb]:"; outputArithmeticType "Output arithmetic type (ufix=0, fix=1, bool=2) [msb ... lsb]:"; show_format "Print format string?"; outputToWorkspace "Output to workspace?"; variablePrefix "Variable name prefix:"; outputToModelAsWell "Output to model as well?"
      mask help:
      | Expands a 'bus' made using a bus_create or Xilinx
      | concat block.
      | The input will be divided into the specified number
      | of outputs with the specified arithmetic types.
      | Divisions are made from most significant bit.
      mask init: same as snap_sys_clk_feng/corr/bus_expand
      settings: AttributesFormatString=7 outputs: uf2.0,uf2.0,uf2.0,uf2.0,uf2.0,uf2.0,uf2.0,
      mask TypeOptions mode: divisions of equal size | divisions of arbitrary size
      mask Callback mode: bus_expand_callback();
      mask Callback outputWidth: bus_expand_callback();
      mask Callback outputToWorkspace: bus_expand_callback();
  debus_wea0 : Subsystem  AncestorBlock=casper_library_flow_control/bus_expand  mask(bus_expand){mode=divisions of equal size, outputNum=7, outputWidth=[1 1 1 1 1 1 1], outputBinaryPt=[0 0 0 0 0 0 0], outputArithmeticType=[2 2 2 2 2 2 2], show_format=on, outputToWorkspace=off, variablePrefix=, outputToModelAsWell=on}
      mask prompts: outputNum "Number of outputs:"; outputWidth "Output width:"; outputBinaryPt "Output binary point position:"; outputArithmeticType "Output arithmetic type (ufix=0, fix=1, bool=2):"; show_format "Print format string?"; outputToWorkspace "Output to workspace?"; variablePrefix "Variable name prefix:"; outputToModelAsWell "Output to model as well?"
      mask help:
      | Expands a 'bus' made using a bus_create or Xilinx
      | concat block.
      | The input will be divided into the specified number
      | of outputs with the specified arithmetic types.
      | Divisions are made from most significant bit.
      mask init: same as snap_sys_clk_feng/corr/bus_expand
      settings: AttributesFormatString=7 outputs: b,b,b,b,b,b,b,
      mask TypeOptions mode: divisions of equal size | divisions of arbitrary size
      mask Callback mode: bus_expand_callback();
      mask Callback outputWidth: bus_expand_callback();
      mask Callback outputToWorkspace: bus_expand_callback();
  debus_web0 : Subsystem  AncestorBlock=casper_library_flow_control/bus_expand  mask(bus_expand){mode=divisions of equal size, outputNum=7, outputWidth=[1 1 1 1 1 1 1], outputBinaryPt=[0 0 0 0 0 0 0], outputArithmeticType=[2 2 2 2 2 2 2], show_format=on, outputToWorkspace=off, variablePrefix=, outputToModelAsWell=on}
      mask prompts: outputNum "Number of outputs:"; outputWidth "Output width:"; outputBinaryPt "Output binary point position:"; outputArithmeticType "Output arithmetic type (ufix=0, fix=1, bool=2):"; show_format "Print format string?"; outputToWorkspace "Output to workspace?"; variablePrefix "Variable name prefix:"; outputToModelAsWell "Output to model as well?"
      mask help:
      | Expands a 'bus' made using a bus_create or Xilinx
      | concat block.
      | The input will be divided into the specified number
      | of outputs with the specified arithmetic types.
      | Divisions are made from most significant bit.
      mask init: same as snap_sys_clk_feng/corr/bus_expand
      settings: AttributesFormatString=7 outputs: b,b,b,b,b,b,b,
      mask TypeOptions mode: divisions of equal size | divisions of arbitrary size
      mask Callback mode: bus_expand_callback();
      mask Callback outputWidth: bus_expand_callback();
      mask Callback outputToWorkspace: bus_expand_callback();
  rep_addra0 : Subsystem  AncestorBlock=casper_library_bus/bus_replicate  mask(bus_replicate){replication=7, csp_latency=4, misc=off, implementation=behavioral}
      mask prompts: replication "replication factor"; csp_latency "latency"; misc "misc support"; implementation "delay implementation"
      mask help: Output bus formed by replicating input bus a number of times
      mask init:
      | bus_replicate_init(gcb, ...
      |     'replication', replication, ...
      |     'csp_latency', csp_latency, ...
      |     'implementation', implementation, ...
      |     'misc', misc);
      mask TypeOptions implementation: core | behavioral
  rep_addrb0 : Subsystem  AncestorBlock=casper_library_bus/bus_replicate  mask(bus_replicate){replication=7, csp_latency=0, misc=off, implementation=core}
      mask prompts: replication "replication factor"; csp_latency "latency"; misc "misc support"; implementation "delay implementation"
      mask help: Output bus formed by replicating input bus a number of times
      mask init:
      | bus_replicate_init(gcb, ...
      |     'replication', replication, ...
      |     'csp_latency', csp_latency, ...
      |     'implementation', implementation, ...
      |     'misc', misc);
      mask TypeOptions implementation: core | behavioral
  rep_wea0 : Subsystem  AncestorBlock=casper_library_bus/bus_replicate  mask(bus_replicate){replication=7, csp_latency=4, misc=off, implementation=core}
      mask prompts: replication "replication factor"; csp_latency "latency"; misc "misc support"; implementation "delay implementation"
      mask help: Output bus formed by replicating input bus a number of times
      mask init:
      | bus_replicate_init(gcb, ...
      |     'replication', replication, ...
      |     'csp_latency', csp_latency, ...
      |     'implementation', implementation, ...
      |     'misc', misc);
      mask TypeOptions implementation: core | behavioral
  rep_web0 : Subsystem  AncestorBlock=casper_library_bus/bus_replicate  mask(bus_replicate){replication=7, csp_latency=0, misc=off, implementation=behavioral}
      mask prompts: replication "replication factor"; csp_latency "latency"; misc "misc support"; implementation "delay implementation"
      mask help: Output bus formed by replicating input bus a number of times
      mask init:
      | bus_replicate_init(gcb, ...
      |     'replication', replication, ...
      |     'csp_latency', csp_latency, ...
      |     'implementation', implementation, ...
      |     'misc', misc);
      mask TypeOptions implementation: core | behavioral
  A : Outport
  B : Outport  Port=2
  wires:
  addrb/1 -> blsbs_slice/1
  addra/1 -> alsbs_slice/1
  blsbs_slice/1 -> rep_addrb0/1(in)
  alsbs_slice/1 -> rep_addra0/1(in)
  dina/1 -> ddina0/1
  wea/1 -> rep_wea0/1(in)
  dinb/1 -> ddinb0/1
  web/1 -> rep_web0/1(in)
  rep_addrb0/1(out) -> debus_addrb0/1(bus_in)
  rep_addra0/1(out) -> debus_addra0/1(bus_in)
  ddina0/1 -> debus_dina0/1(bus_in)
  rep_wea0/1(out) -> debus_wea0/1(bus_in)
  ddinb0/1 -> debus_dinb0/1(bus_in)
  rep_web0/1(out) -> debus_web0/1(bus_in)
  debus_addra0/1(msb_out7) -> bram0_0/1
  debus_dina0/1(msb_out7) -> bram0_0/2
  debus_wea0/1(msb_out7) -> bram0_0/3
  debus_addrb0/1(msb_out7) -> bram0_0/4
  debus_dinb0/1(msb_out7) -> bram0_0/5
  debus_web0/1(msb_out7) -> bram0_0/6
  debus_addra0/2(out6) -> bram0_1/1
  debus_dina0/2(out6) -> bram0_1/2
  debus_wea0/2(out6) -> bram0_1/3
  debus_addrb0/2(out6) -> bram0_1/4
  debus_dinb0/2(out6) -> bram0_1/5
  debus_web0/2(out6) -> bram0_1/6
  debus_addra0/3(out5) -> bram0_2/1
  debus_dina0/3(out5) -> bram0_2/2
  debus_wea0/3(out5) -> bram0_2/3
  debus_addrb0/3(out5) -> bram0_2/4
  debus_dinb0/3(out5) -> bram0_2/5
  debus_web0/3(out5) -> bram0_2/6
  debus_addra0/4(out4) -> bram0_3/1
  debus_dina0/4(out4) -> bram0_3/2
  debus_wea0/4(out4) -> bram0_3/3
  debus_addrb0/4(out4) -> bram0_3/4
  debus_dinb0/4(out4) -> bram0_3/5
  debus_web0/4(out4) -> bram0_3/6
  debus_addra0/5(out3) -> bram0_4/1
  debus_dina0/5(out3) -> bram0_4/2
  debus_wea0/5(out3) -> bram0_4/3
  debus_addrb0/5(out3) -> bram0_4/4
  debus_dinb0/5(out3) -> bram0_4/5
  debus_web0/5(out3) -> bram0_4/6
  debus_addra0/6(out2) -> bram0_5/1
  debus_dina0/6(out2) -> bram0_5/2
  debus_wea0/6(out2) -> bram0_5/3
  debus_addrb0/6(out2) -> bram0_5/4
  debus_dinb0/6(out2) -> bram0_5/5
  debus_web0/6(out2) -> bram0_5/6
  debus_addra0/7(lsb_out1) -> bram0_6/1
  debus_dina0/7(lsb_out1) -> bram0_6/2
  debus_wea0/7(lsb_out1) -> bram0_6/3
  debus_addrb0/7(lsb_out1) -> bram0_6/4
  debus_dinb0/7(lsb_out1) -> bram0_6/5
  debus_web0/7(lsb_out1) -> bram0_6/6
  bram0_0/1 -> A_bussify0/1(in1)
  bram0_0/2 -> B_bussify0/1(in1)
  bram0_1/1 -> A_bussify0/2(in2)
  bram0_1/2 -> B_bussify0/2(in2)
  bram0_2/1 -> A_bussify0/3(in3)
  bram0_2/2 -> B_bussify0/3(in3)
  bram0_3/1 -> A_bussify0/4(in4)
  bram0_3/2 -> B_bussify0/4(in4)
  bram0_4/1 -> A_bussify0/5(in5)
  bram0_4/2 -> B_bussify0/5(in5)
  bram0_5/1 -> A_bussify0/6(in6)
  bram0_5/2 -> B_bussify0/6(in6)
  bram0_6/1 -> A_bussify0/7(in7)
  bram0_6/2 -> B_bussify0/7(in7)
  A_bussify0/1(bus_out) -> A/1
  B_bussify0/1(bus_out) -> B/1

== system snap_sys_clk_feng/chan_reorder/reorder3/edge_detect ==
  in : Inport
  Delay : xbsIndex_r4/Delay  rst=off  infoeditControl=Selection of Reset will increase slice count due to use of real FFs and instead of SRLs  en=off  latency=1  reg_retiming=off  dbl_ovrd=off  block_type=delay
      settings: xl_area=[0, 0, 0, 0, 0, 0, 0]
  Inverter : xbsIndex_r4/Inverter  en=off  latency=0  dbl_ovrd=off  block_type=inv
      settings: xl_area=[0, 0, 0, 0, 0, 0, 0]
  edge_op : xbsIndex_r4/Logical  logical_function=AND  inputs=2  en=off  latency=0  precision=Full  arith_type=Unsigned  n_bits=8  bin_pt=2  align_bp=on  dbl_ovrd=off  block_type=logical
      settings: xl_area=[0, 0, 0, 0, 0, 0, 0]
  out : Outport
  wires:
  Inverter/1 -> edge_op/1
  edge_op/1 -> out/1
  in/1 -> Inverter/1, Delay/1
  Delay/1 -> edge_op/2
